simulink model "ac_power"  (R2026a)
settings: Solver=ode1  StopTime=0.02  FixedStep=0.02/(n-1)
values from neighbouring files (symbols this model uses):
  n = 100    [ac_power_signals.m]
libraries: eeRmsMeasurement x1
settings Model: Creator=HAKAN SARI  LastModifiedBy=HAKAN SARI

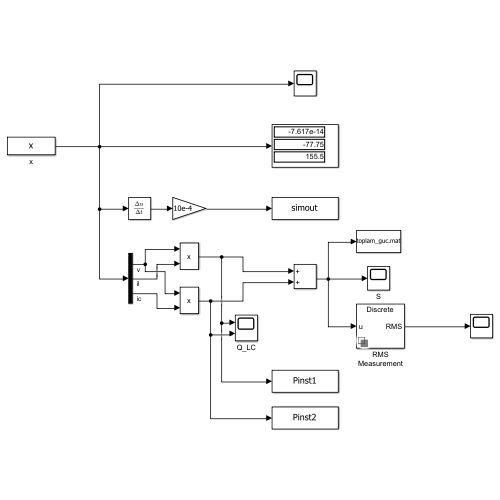
[thumbnail: Simulink's stored preview of the top-level diagram]
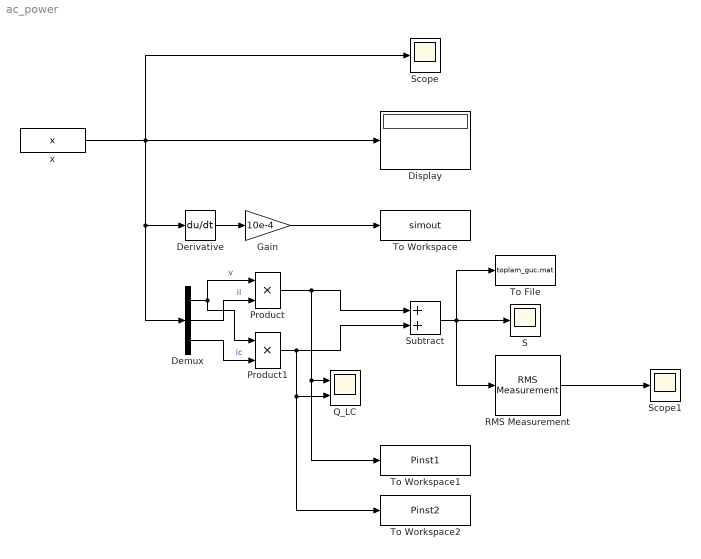
== system ac_power ==
  Demux : Demux  Outputs=3
  Derivative : Derivative
  Display : Display
  Gain : Gain  Gain=10e-4
  Product : Product
  Product1 : Product
  Q_LC : Scope  NumInputPorts=2
      settings: MaximizeAxes=On  ActiveDisplayYMinimum=-76148.549016609541  ActiveDisplayYMaximum=97089.259786468217  DataLoggingVariableName=Q_LC
  RMS Measurement : eeRmsMeasurement/RMS Measurement  LabelModeActiveChoice=Total  F=50  SpecifyHarmonics=off  K=[0 1 2]  Ts=0.02/(n-1)
      settings: LibrarySourceBlock=|
      | ee_sl_lib/Measurements/RMS
      | Measurement
  S : Scope
      settings: ActiveDisplayYMinimum=-9280.7971997490968  ActiveDisplayYMaximum=51162.218739466451
  Scope : Scope
      settings: MaximizeAxes=On  ActiveDisplayYMinimum=-388.70106713321894  ActiveDisplayYMaximum=388.70106713321894
  Scope1 : Scope
      settings: ActiveDisplayYMinimum=-1  ActiveDisplayYMaximum=1  DataLoggingVariableName=ScopeData2
  Subtract : Sum
  To File : ToFile  Filename=toplam_guc.mat
  To Workspace : ToWorkspace  VariableName=simout  SaveFormat=Timeseries  SampleTime=-1
  To Workspace1 : ToWorkspace  VariableName=Pinst1  SampleTime=-1
      settings: Save2DSignal=2-D array (concatenate along first dimension)
  To Workspace2 : ToWorkspace  VariableName=Pinst2  SampleTime=-1
      settings: Save2DSignal=2-D array (concatenate along first dimension)
  x : FromWorkspace  VariableName=x
  wires:
  x/1 -> Scope/1, Display/1, Demux/1, Derivative/1
  Derivative/1 -> Gain/1
  Gain/1 -> To Workspace/1
  RMS Measurement/1 -> Scope1/1
  Product/1 -> To Workspace1/1, Q_LC/1, Subtract/1
  Product1/1 -> To Workspace2/1, Q_LC/2, Subtract/2
  Subtract/1 -> To File/1, S/1, RMS Measurement/1
  Demux/3 -> Product1/2  "ic"
  Demux/2 -> Product/2  "il"
  Demux/1 -> Product1/1, Product/1  "v"
